simulink model "bancDEssay"  (R2024a)
settings: Solver=VariableStepAuto  StartTime=0.0  StopTime=10.0  RelTol=1e-3
libraries: spsSeriesRLCBranchLib x10, spsVoltageMeasurementLib x6, spsDiodeLib x5, spsGroundLib x4, spsCurrentMeasurementLib x2, spsDCMachineLib x1, spsMosfetLib x1, spspowerguiLib x1
settings Model: Creator=nadh6692  LastModifiedBy=nadh6692

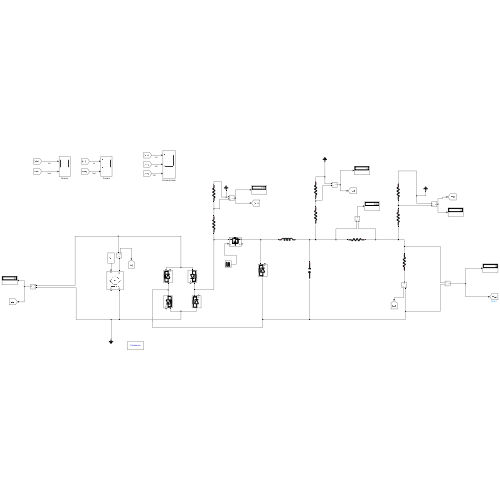
[thumbnail: Simulink's stored preview of the top-level diagram]
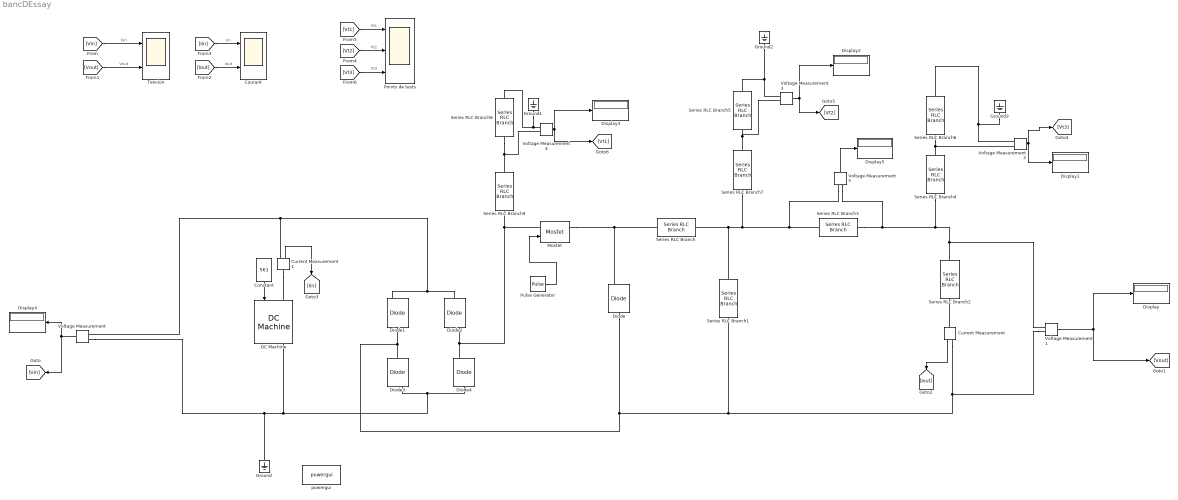
== system bancDEssay ==
  Constant : Constant  Value=561
  Courant : Scope  NumInputPorts=2
  Current Measurement : spsCurrentMeasurementLib/Current Measurement  PhasorSimulation=off  OutputType=Complex  PSBequivalent=0
  Current Measurement1 : spsCurrentMeasurementLib/Current Measurement  PhasorSimulation=off  OutputType=Complex  PSBequivalent=0
  DC Machine : spsDCMachineLib/DC Machine  PresetModel=No  MechanicalLoad=Speed w  FieldType=Permanent magnet  ShowDetailedParameters=on  MeasurementBus=off  RLa="[ 0.00002  0.004]"  RLf="[ 240  120]"  Laf=1.8  MachineConstant=Back-emf constant (V/rpm)  Ke=0.0112  Kt=1.8  J=0.00002  Bm=0.00006  Tf=0  w0=1  Ifinit=1  TsPowergui=0  TsBlock=-1
  Diode{,1..4} (5 alike) : spsDiodeLib/Diode  Ron=0.001  Lon=0  Vf=0.8  IC=0  UseSnubber=0  Rs=500  Cs=250e-9  Measurements=on
  Display{,1..5} (6 alike) : Display
  Ground{,1..3} (4 alike) : spsGroundLib/Ground  LConnTagsString=a
  Mosfet : spsMosfetLib/Mosfet  Ron=0.1  Lon=0  Rd=0.01  Vfd=0  IC=0  Rs=1e5  Cs=inf  Measurements=on
  Points de tests : Scope  NumInputPorts=3
  Pulse Generator : DiscretePulseGenerator  PulseType=Time based  Period=0.002  PulseWidth=33
  Series RLC Branch : spsSeriesRLCBranchLib/Series RLC Branch  LConnTagsString=__new0  RConnTagsString=__new0  BranchType=L  Resistance=1  Inductance=0.03265  SetiL0=off  InitialCurrent=0  Capacitance=1e-6  Setx0=off  InitialVoltage=0  Measurements=None
  Series RLC Branch1 : spsSeriesRLCBranchLib/Series RLC Branch  LConnTagsString=__new0  RConnTagsString=__new0  BranchType=C  Resistance=1  Inductance=1e-3  SetiL0=off  InitialCurrent=0  Capacitance=0.00153  Setx0=off  InitialVoltage=0  Measurements=None
  Series RLC Branch2 : spsSeriesRLCBranchLib/Series RLC Branch  LConnTagsString=__new0  RConnTagsString=__new0  BranchType=R  Resistance=6  Inductance=1e-3  SetiL0=off  InitialCurrent=0  Capacitance=1e-6  Setx0=off  InitialVoltage=0  Measurements=None
  Series RLC Branch3 : spsSeriesRLCBranchLib/Series RLC Branch  LConnTagsString=__new0  RConnTagsString=__new0  BranchType=R  Resistance=1  Inductance=1e-3  SetiL0=off  InitialCurrent=0  Capacitance=1e-6  Setx0=off  InitialVoltage=0  Measurements=None
  Series RLC Branch4 : spsSeriesRLCBranchLib/Series RLC Branch  LConnTagsString=__new0  RConnTagsString=__new0  BranchType=R  Resistance=9000000  Inductance=1e-3  SetiL0=off  InitialCurrent=0  Capacitance=1e-6  Setx0=off  InitialVoltage=0  Measurements=None
  Series RLC Branch5 : spsSeriesRLCBranchLib/Series RLC Branch  LConnTagsString=__new0  RConnTagsString=__new0  BranchType=R  Resistance=1000000  Inductance=1e-3  SetiL0=off  InitialCurrent=0  Capacitance=1e-6  Setx0=off  InitialVoltage=0  Measurements=None
  Series RLC Branch6 : spsSeriesRLCBranchLib/Series RLC Branch  LConnTagsString=__new0  RConnTagsString=__new0  BranchType=R  Resistance=1000000  Inductance=1e-3  SetiL0=off  InitialCurrent=0  Capacitance=1e-6  Setx0=off  InitialVoltage=0  Measurements=None
  Series RLC Branch7 : spsSeriesRLCBranchLib/Series RLC Branch  LConnTagsString=__new0  RConnTagsString=__new0  BranchType=R  Resistance=9000000  Inductance=1e-3  SetiL0=off  InitialCurrent=0  Capacitance=1e-6  Setx0=off  InitialVoltage=0  Measurements=None
  Series RLC Branch8 : spsSeriesRLCBranchLib/Series RLC Branch  LConnTagsString=__new0  RConnTagsString=__new0  BranchType=R  Resistance=100000  Inductance=1e-3  SetiL0=off  InitialCurrent=0  Capacitance=1e-6  Setx0=off  InitialVoltage=0  Measurements=None
  Series RLC Branch9 : spsSeriesRLCBranchLib/Series RLC Branch  LConnTagsString=__new0  RConnTagsString=__new0  BranchType=R  Resistance=9000000  Inductance=1e-3  SetiL0=off  InitialCurrent=0  Capacitance=1e-6  Setx0=off  InitialVoltage=0  Measurements=None
  Tension : Scope  NumInputPorts=2
  Voltage Measurement{,1..5} (6 alike) : spsVoltageMeasurementLib/Voltage Measurement  PhasorSimulation=off  OutputType=Complex  PSBequivalent=0
  powergui : spspowerguiLib/powergui  Priority=1  SimulationMode=Continuous  SampleTime=50e-6  frequency=60  Iterations=50  frequencyindice=0  Pbase=100e6  ErrMax=1e-4  UnitsV=kV  UnitsW=MW  buscounter=0  FunctionMessages=off  echomessages=off  EnableUseOfTLC=off  CurrentSourceSwitches=off  DisableSnubberDevices=off  DisableRonSwitches=off  DisableVfSwitches=off  DisplayEquations=off  AutomaticDiscreteSolvers=off  SolverType=Tustin/Backward Euler (TBE)  Interpol=off  ExternalGateDelay=off  methode=off  Ts=100  x0status=blocks  SPID=on  SwTol=0  HookPort=off  NonlinearTolerance=1e-4  nMaxIteration=100  ContinueOnMaxIteration=off  RestoreLinks=warning  ResistiveCurrentMeasurement=off  Frange=[0:2:500]  Ylog=off  Xlog=on  ShowGrid=off  save=off  variable=ZData  structure=0  ZoomFFT=off  StartTime=0.0  cycles=1  DisplayStyle=1  fundamental=60  FreqAxis=off  MaxFrequency=1000  frequencyindicesteady=1  RmsSteady=1  display=off
  wires:
  Voltage Measurement/1 -> Display4/1, [Vin]
  [Vin] -> Tension/1  "Vin"
  Voltage Measurement1/1 -> Display/1, [Vout]
  [Vout] -> Tension/2  "Vout"
  [Iout] -> Courant/2  "Iout"
  Current Measurement1/1 -> [Iin]
  [Iin] -> Courant/1  "Iin"
  Pulse Generator/1 -> Mosfet/1
  Current Measurement/1 -> [Iout]
  Voltage Measurement2/1 -> Display1/1, [Vt3]
  Voltage Measurement3/1 -> [Vt2], Display2/1
  Voltage Measurement4/1 -> Display3/1, [Vt1]
  [Vt1] -> Points de tests/1  "Vt1"
  [Vt2] -> Points de tests/2  "Vt2"
  [Vt3] -> Points de tests/3  "Vt3"
  Constant/1 -> DC Machine/1
  Voltage Measurement5/1 -> Display5/1
  connections:
  Mosfet/RConn1 -- Series RLC Branch/LConn1 -- Diode/RConn1
  Series RLC Branch3/RConn1 -- Series RLC Branch7/RConn1 -- Series RLC Branch/RConn1 -- Series RLC Branch1/LConn1 -- Voltage Measurement5/LConn1
  Current Measurement/LConn1 -- Series RLC Branch2/LConn1
  Series RLC Branch2/RConn1 -- Voltage Measurement5/LConn2 -- Series RLC Branch3/LConn1 -- Series RLC Branch4/RConn1 -- Voltage Measurement1/LConn1
  Series RLC Branch6/RConn1 -- Series RLC Branch4/LConn1 -- Voltage Measurement2/LConn1
  Series RLC Branch5/RConn1 -- Series RLC Branch7/LConn1 -- Voltage Measurement3/LConn1
  Series RLC Branch8/RConn1 -- Series RLC Branch9/LConn1 -- Voltage Measurement4/LConn1
  Current Measurement1/LConn1 -- DC Machine/LConn1
  Voltage Measurement4/LConn2 -- Series RLC Branch8/LConn1 -- Ground1/LConn1
  Voltage Measurement3/LConn2 -- Ground2/LConn1 -- Series RLC Branch5/LConn1
  Series RLC Branch6/LConn1 -- Ground3/LConn1 -- Voltage Measurement2/LConn2
  Diode4/RConn1 -- Mosfet/LConn1 -- Series RLC Branch9/RConn1 -- Diode2/RConn1
  Voltage Measurement1/LConn2 -- Diode/LConn1 -- Diode1/LConn1 -- Diode3/LConn1 -- Series RLC Branch1/RConn1 -- Current Measurement/RConn1
  Current Measurement1/RConn1 -- Voltage Measurement/LConn1 -- Diode2/LConn1 -- Diode1/RConn1
  Voltage Measurement/LConn2 -- Ground/LConn1 -- DC Machine/RConn1 -- Diode3/RConn1 -- Diode4/LConn1
